simulink library "Lib_Piccolo"  (R2018b)
settings: Solver=VariableStepAuto  StartTime=0.0  StopTime=10.0  RelTol=1e-3
values from neighbouring files (symbols this model uses):
  AccelErrInt2Brakes = 0.15    [SimulationControlConfig16P.m]    (also in SimulationControlConfig16P_LEGACY.m; SimulationControlConfigTAILLESS.m = 0.2; SimulationControlConfigUTAIL.m = 0.2)
  AileronMax = 25    [SimulationControlConfig16P.m]    (also in SimulationControlConfig16P_LEGACY.m; SimulationControlConfigTAILLESS.m; SimulationControlConfigUTAIL.m)
  AileronPower = 0.00268    [SimulationControlConfig16P.m]    (also in SimulationControlConfig16P_LEGACY.m; SimulationControlConfigTAILLESS.m; SimulationControlConfigUTAIL.m)
  AileronSurfaceMax = 45    [SimulationControlConfig16P.m]    (also in SimulationControlConfig16P_LEGACY.m)
  AileronTrim = 0    [SimulationControlConfig16P.m]    (also in SimulationControlConfig16P_LEGACY.m; SimulationControlConfigTAILLESS.m; SimulationControlConfigUTAIL.m)
  Alt = 1000 + TerrainHeight    [SimulationStateConfig.m]
  AltCruise_m = testPlans(testIndx).terrainElevation * 0.3048 + 200    [SimulationControlConfig16P.m]    (also in SimulationControlConfigTAILLESS.m = 1083; SimulationControlConfigUTAIL.m = testPlans(testIndx).terrainElevation * 0.3048 + 152)
  AltitudeRate2PitchCmdIntegratorInit = 0.1    [SimulationControlPre.m]
  AltMax = 10000    [SimulationControlConfig16P.m]    (also in SimulationControlConfig16P_LEGACY.m; SimulationControlConfigTAILLESS.m; SimulationControlConfigUTAIL.m)
  AltMaxAccel = 1.25    [SimulationControlConfig16P.m]    (also in SimulationControlConfig16P_LEGACY.m = 0.9; SimulationControlConfigTAILLESS.m = 1.7; SimulationControlConfigUTAIL.m = 2)
  AltMin = 0    [SimulationControlConfig16P.m]    (also in SimulationControlConfig16P_LEGACY.m; SimulationControlConfigTAILLESS.m; SimulationControlConfigUTAIL.m)
  AltRateCmd2Pitch = 0.50    (= 0.5)    [SimulationControlConfig16P.m]    (also in SimulationControlConfig16P_LEGACY.m = 0.6; SimulationControlConfigTAILLESS.m = 0.2; SimulationControlConfigUTAIL.m = 0.3)
  AltRateError2Pitch = 0.40    (= 0.4)    [SimulationControlConfig16P.m]    (also in SimulationControlConfig16P_LEGACY.m; SimulationControlConfigTAILLESS.m = 0.55; SimulationControlConfigUTAIL.m = 0.55)
  AltRateErrorInt2Pitch = 0.50    (= 0.5)    [SimulationControlConfig16P.m]    (also in SimulationControlConfig16P_LEGACY.m = 0.45; SimulationControlConfigTAILLESS.m; SimulationControlConfigUTAIL.m = 0.75)
  AltRateLpfCutOff = 3    [SimulationControlConfig16P.m]    (also in SimulationControlConfig16P_LEGACY.m; SimulationControlConfigTAILLESS.m = 2; SimulationControlConfigUTAIL.m = 2)
  AutoNosegear2Rudder = 26    [SimulationControlConfig16P.m]    (also in SimulationControlConfig16P_LEGACY.m; SimulationControlConfigTAILLESS.m = 25.2; SimulationControlConfigUTAIL.m = 14)
  b = 5.54    [SimulationControlConfig16P.m]    (also in SimulationControlConfig16P_LEGACY.m; SimulationControlConfigTAILLESS.m = 2.37; SimulationControlConfigUTAIL.m = 2.37)
  Bank2AileronIntegratorInit = 0    [SimulationControlPre.m]
  BankMax_User = BankMax_User/180*pi    (= 0.523598775598)    [SimulationControlConfig16P.m]    (also in SimulationControlConfig16P_LEGACY.m; SimulationControlConfigTAILLESS.m = 0.610865238198; SimulationControlConfigUTAIL.m = 0.628318530718)
  baseLegFlaps = 20    [SimulationControlConfig16P.m]    (also in SimulationControlConfig16P_LEGACY.m = 0; SimulationControlConfigTAILLESS.m = 15; SimulationControlConfigUTAIL.m = 10)
  C = GeneticOpt.C    [SimulationCostFunction.m]
  c = Sw/b    (= 0.841696750903)    [SimulationControlConfig16P.m]    (also in SimulationControlConfig16P_LEGACY.m; SimulationControlConfigTAILLESS.m = 0.354008438819; SimulationControlConfigUTAIL.m = 0.354008438819)
  cell2WheelFactorMG = 5.98    [SimulationSensorConfig16P_LEGACY.m]
  cell2WheelFactorNG = 1    [SimulationSensorConfig16P_LEGACY.m]
  cellSatMaxMG = 15000    [SimulationSensorConfig16P.m]    (also in SimulationSensorConfig16P_LEGACY.m; SimulationSensorConfigTAILLESS7P.m; SimulationSensorConfigUTAIL7P.m)
  cellSatMaxNG = 1000    [SimulationSensorConfig16P.m]    (also in SimulationSensorConfig16P_LEGACY.m; SimulationSensorConfigTAILLESS7P.m; SimulationSensorConfigUTAIL7P.m)
  cellSatMinMG = -15000    [SimulationSensorConfig16P.m]    (also in SimulationSensorConfig16P_LEGACY.m; SimulationSensorConfigTAILLESS7P.m; SimulationSensorConfigUTAIL7P.m)
  cellSatMinNG = -1000    [SimulationSensorConfig16P.m]    (also in SimulationSensorConfig16P_LEGACY.m; SimulationSensorConfigTAILLESS7P.m; SimulationSensorConfigUTAIL7P.m)
  CL_Limit = CL_Max    (= 0.54)    [SimulationControlConfig16P.m]    (also in SimulationControlConfig16P_LEGACY.m; SimulationControlConfigTAILLESS.m; SimulationControlConfigUTAIL.m = 0.53)
  CL_Max = 0.54    [SimulationControlConfig16P.m]    (also in SimulationControlConfig16P_LEGACY.m; SimulationControlConfigTAILLESS.m; SimulationControlConfigUTAIL.m = 0.53)
  CL_Max_Nom = 0.465    [SimulationControlConfig16P.m]    (also in SimulationControlConfig16P_LEGACY.m; SimulationControlConfigTAILLESS.m = 0.39; SimulationControlConfigUTAIL.m)
  CL_Min = 0    [SimulationControlConfig16P.m]    (also in SimulationControlConfig16P_LEGACY.m; SimulationControlConfigTAILLESS.m; SimulationControlConfigUTAIL.m)
  ClimbMaxFraction = 0.35    [SimulationControlConfig16P.m]    (also in SimulationControlConfig16P_LEGACY.m = 0.24; SimulationControlConfigTAILLESS.m = 0.19; SimulationControlConfigUTAIL.m = 0.21)
  ClimboutMaxBank = 7.0    (= 7)    [SimulationControlConfig16P.m]    (also in SimulationControlConfig16P_LEGACY.m; SimulationControlConfigTAILLESS.m = 5; SimulationControlConfigUTAIL.m)
  ClimboutTimer = 7.0    (= 7)    [SimulationControlConfig16P.m]    (also in SimulationControlConfig16P_LEGACY.m; SimulationControlConfigTAILLESS.m; SimulationControlConfigUTAIL.m)
  dCl_per_dFlap = 0.005581818    [SimulationControlConfig16P.m]    (also in SimulationControlConfig16P_LEGACY.m = 0; SimulationControlConfigTAILLESS.m = 0; SimulationControlConfigUTAIL.m = 0)
  DecelerationCmd = 3.1    [SimulationControlConfig16P.m]    (also in SimulationControlConfig16P_LEGACY.m; SimulationControlConfigTAILLESS.m = 0.1; SimulationControlConfigUTAIL.m = 0.1)
  DeRotateLogicEndTimer = abs((NoseDownLimit_Deg-1)/DeRotateRamp_Dps)    [SimulationControlConfig16P.m]    (also in SimulationControlConfig16P_LEGACY.m; SimulationControlConfigTAILLESS.m; SimulationControlConfigUTAIL.m)
  DeRotateLogicHoldNoseUpTimer = 0.1    [SimulationControlConfig16P.m]    (also in SimulationControlConfig16P_LEGACY.m; SimulationControlConfigTAILLESS.m; SimulationControlConfigUTAIL.m)
  DeRotateLogicTimerTimeout = 2    [SimulationControlConfig16P.m]    (also in SimulationControlConfig16P_LEGACY.m; SimulationControlConfigTAILLESS.m; SimulationControlConfigUTAIL.m)
  DeRotateLowerCmdSaturation = 0    [SimulationControlConfig16P.m]    (also in SimulationControlConfig16P_LEGACY.m; SimulationControlConfigTAILLESS.m; SimulationControlConfigUTAIL.m)
  DeRotateRamp_Dps = 3    [SimulationControlConfig16P.m]    (also in SimulationControlConfig16P_LEGACY.m; SimulationControlConfigTAILLESS.m = 8; SimulationControlConfigUTAIL.m = 8)
  DeRotateUpperCmdSaturation = 7    [SimulationControlConfig16P.m]    (also in SimulationControlConfig16P_LEGACY.m; SimulationControlConfigTAILLESS.m; SimulationControlConfigUTAIL.m)
  DescentMaxFraction = 0.22    [SimulationControlConfig16P.m]    (also in SimulationControlConfig16P_LEGACY.m = 0.2; SimulationControlConfigTAILLESS.m = 0.17; SimulationControlConfigUTAIL.m = 0.17)
  DesktopSimTerrainOffset_m = 0.406    [SimulationAircraftConfig.m]
  downwindFlaps = 0    [SimulationControlConfig16P.m]    (also in SimulationControlConfig16P_LEGACY.m; SimulationControlConfigTAILLESS.m; SimulationControlConfigUTAIL.m)
  DP_init = 0.5*1.225*V_init^2    [SimulationControlConfig16P.m]    (also in SimulationControlConfig16P_LEGACY.m; SimulationControlConfigTAILLESS.m; SimulationControlConfigUTAIL.m)
  dscNoiseMG = 1    [SimulationSensorConfig16P_LEGACY.m]
  dscNoiseNG = 0.25    [SimulationSensorConfig16P_LEGACY.m]
  DSCnumBits = 24    [SimulationSensorConfig16P.m]    (also in SimulationSensorConfig16P_LEGACY.m; SimulationSensorConfigTAILLESS7P.m; SimulationSensorConfigUTAIL7P.m)
  DSCRangeMaxMG = 15000    [SimulationSensorConfig16P.m]    (also in SimulationSensorConfig16P_LEGACY.m; SimulationSensorConfigTAILLESS7P.m; SimulationSensorConfigUTAIL7P.m)
  DSCRangeMaxNG = 1000    [SimulationSensorConfig16P.m]    (also in SimulationSensorConfig16P_LEGACY.m; SimulationSensorConfigTAILLESS7P.m; SimulationSensorConfigUTAIL7P.m)
  DSCRangeMinMG = -15000    [SimulationSensorConfig16P.m]    (also in SimulationSensorConfig16P_LEGACY.m; SimulationSensorConfigTAILLESS7P.m; SimulationSensorConfigUTAIL7P.m)
  DSCRangeMinNG = -1000    [SimulationSensorConfig16P.m]    (also in SimulationSensorConfig16P_LEGACY.m; SimulationSensorConfigTAILLESS7P.m; SimulationSensorConfigUTAIL7P.m)
  dt = DLLSim.dt    [SimulationTimeStep.m]    (also in SimulationTrim.m = 0.02)
  EarlyTouchdownThreshold = 3.0    (= 3)    [SimulationControlConfig16P.m]    (also in SimulationControlConfig16P_LEGACY.m; SimulationControlConfigTAILLESS.m = 2.2; SimulationControlConfigUTAIL.m = 2.5)
  ElevatorDeflectionRate = 15    [SimulationControlConfig16P.m]    (also in SimulationControlConfig16P_LEGACY.m = 12; SimulationControlConfigTAILLESS.m = 10; SimulationControlConfigUTAIL.m = 12)
  ElevatorMax = 25    [SimulationControlConfig16P.m]    (also in SimulationControlConfig16P_LEGACY.m; SimulationControlConfigTAILLESS.m; SimulationControlConfigUTAIL.m)
  ElevatorPower = -0.002209    [SimulationControlConfig16P.m]    (also in SimulationControlConfig16P_LEGACY.m; SimulationControlConfigTAILLESS.m = -0.002956; SimulationControlConfigUTAIL.m = -0.00205983)
  ElevatorTrim = -3.5    [SimulationControlConfig16P.m]    (also in SimulationControlConfig16P_LEGACY.m; SimulationControlConfigTAILLESS.m = -6; SimulationControlConfigUTAIL.m = -8)
  elevonBias = 0    [SimulationControlConfig16P.m]    (also in SimulationControlConfig16P_LEGACY.m; SimulationControlConfigTAILLESS.m; SimulationControlConfigUTAIL.m)
  Enable_TAS_Protection = 0    [SimulationControlConfig16P.m]    (also in SimulationControlConfig16P_LEGACY.m; SimulationControlConfigTAILLESS.m; SimulationControlConfigUTAIL.m)
  EnableCrossTrackAbort = 1    [SimulationControlConfig16P.m]    (also in SimulationControlConfigTAILLESS.m; SimulationControlConfigUTAIL.m)
  EnergyBandwidth = 0.02    [SimulationControlConfig16P.m]    (also in SimulationControlConfig16P_LEGACY.m; SimulationControlConfigTAILLESS.m = 0.06; SimulationControlConfigUTAIL.m = 0.06)
  EngineLhFuelCut = 0    [SimulationAircraftConfig.m]
  EngineRhFuelCut = 0    [SimulationAircraftConfig.m]
  FastThrottleRate = 0.075    [SimulationControlConfig16P.m]    (also in SimulationControlConfig16P_LEGACY.m = 0.05; SimulationControlConfigTAILLESS.m = 0.1; SimulationControlConfigUTAIL.m = 0.1)
  FilterWarmUpTime = 2    [SimulationSensorConfig16P.m]    (also in SimulationSensorConfig16P_LEGACY.m; SimulationSensorConfigTAILLESS7P.m; SimulationSensorConfigUTAIL7P.m)
  finalApproachFlaps = 20    [SimulationControlConfig16P.m]    (also in SimulationControlConfig16P_LEGACY.m = 0; SimulationControlConfigTAILLESS.m = 22; SimulationControlConfigUTAIL.m = 10)
  FinalDescentSlope_Deg = testPlans(testIndx).descentSlope    [SimulationControlConfig16P.m]    (also in SimulationControlConfig16P_LEGACY.m; SimulationControlConfigTAILLESS.m; SimulationControlConfigUTAIL.m)
  flapMax = 0    [SimulationControlConfig16P.m]    (also in SimulationControlConfig16P_LEGACY.m; SimulationControlConfigTAILLESS.m; SimulationControlConfigUTAIL.m)
  flapRate = 7.5    [SimulationControlConfig16P.m]    (also in SimulationControlConfig16P_LEGACY.m; SimulationControlConfigTAILLESS.m = 6.6; SimulationControlConfigUTAIL.m)
  FlareHeight = 5    [SimulationControlConfig16P.m]    (also in SimulationControlConfig16P_LEGACY.m = 4.8; SimulationControlConfigTAILLESS.m = 2.5; SimulationControlConfigUTAIL.m = 2)
  FlareVerticalRate_mps = -0.4    [SimulationControlConfig16P.m]    (also in SimulationControlConfig16P_LEGACY.m = -0.5; SimulationControlConfigTAILLESS.m = -0.15; SimulationControlConfigUTAIL.m = -0.15)
  Fp_Aileron = 0.55*2*pi*RollRateLpfCutoff*dt    [SimulationControlConfig16P.m]    (also in SimulationControlConfig16P_LEGACY.m; SimulationControlConfigTAILLESS.m; SimulationControlConfigUTAIL.m)
  Fp_Alt = 0.55*AltBandwidth    (= 0.099)    [SimulationControlConfig16P.m]    (also in SimulationControlConfig16P_LEGACY.m; SimulationControlConfigTAILLESS.m = 0.587477826221; SimulationControlConfigUTAIL.m = 0.69115038379)
  Fp_AltRate = 0.55*2*pi*AltRateLpfCutOff*dt    [SimulationControlConfig16P.m]    (also in SimulationControlConfig16P_LEGACY.m; SimulationControlConfigTAILLESS.m; SimulationControlConfigUTAIL.m)
  Fp_Elevator = 0.55*2*pi*PitchRateLpfCutoff*dt    [SimulationControlConfig16P.m]    (also in SimulationControlConfig16P_LEGACY.m; SimulationControlConfigTAILLESS.m; SimulationControlConfigUTAIL.m)
  Fp_Energy = 0.55*2*pi*EnergyBandwidth    (= 0.069115038379)    [SimulationControlConfig16P.m]    (also in SimulationControlConfig16P_LEGACY.m; SimulationControlConfigTAILLESS.m = 0.207345115137; SimulationControlConfigUTAIL.m = 0.207345115137)
  Fp_Energy2 = 0.55*2*pi*EnergyBandwidth*dt    [SimulationControlConfig16P.m]    (also in SimulationControlConfig16P_LEGACY.m; SimulationControlConfigTAILLESS.m; SimulationControlConfigUTAIL.m)
  Fp_Pitch = 0.55*2*pi*PitchBandwidth    (= 2.76460153516)    [SimulationControlConfig16P.m]    (also in SimulationControlConfig16P_LEGACY.m = 3.11017672705; SimulationControlConfigTAILLESS.m = 3.80132711084; SimulationControlConfigUTAIL.m = 2.41902634326)
  Fp_Pitch_2 = 0.55*2*pi*PitchBandwidth*dt    [SimulationControlConfig16P.m]    (also in SimulationControlConfig16P_LEGACY.m; SimulationControlConfigTAILLESS.m; SimulationControlConfigUTAIL.m)
  Fp_Roll = RollBandwidth^2    (= 1)    [SimulationControlConfig16P.m]    (also in SimulationControlConfig16P_LEGACY.m = 1.44; SimulationControlConfigTAILLESS.m; SimulationControlConfigUTAIL.m)
  Fp_Rudder = 0.55*2*pi*YawRateLpfCutoff*dt    [SimulationControlConfig16P.m]    (also in SimulationControlConfig16P_LEGACY.m; SimulationControlConfigTAILLESS.m; SimulationControlConfigUTAIL.m)
  Fp_TAS = 0.55*2*pi*TASBandwidth    (= 0.103672557568)    [SimulationControlConfig16P.m]    (also in SimulationControlConfig16P_LEGACY.m; SimulationControlConfigTAILLESS.m = 0.172787595947; SimulationControlConfigUTAIL.m = 0.172787595947)
  Fp_TAS_Filter = 2*pi*TasLpfCutoff*dt    [SimulationControlConfig16P.m]    (also in SimulationControlConfig16P_LEGACY.m; SimulationControlConfigTAILLESS.m; SimulationControlConfigUTAIL.m)
  Fp_Turn = 0.55*2*pi*TurnErrLPFcutoff    (= 0.0345575191895)    [SimulationControlConfig16P.m]    (also in SimulationControlConfig16P_LEGACY.m; SimulationControlConfigTAILLESS.m = 0.172787595947; SimulationControlConfigUTAIL.m = 0.172787595947)
  Fp_TurnDerr = 0.55*2*pi*TurnDerivativeLPFcutoff    (= 0.0345575191895)    [SimulationControlConfig16P.m]    (also in SimulationControlConfig16P_LEGACY.m; SimulationControlConfigTAILLESS.m = 0.172787595947; SimulationControlConfigUTAIL.m = 0.172787595947)
  FTV = 3    [SimulationAircraftConfig.m]
  ftvStaticPositionError = 1/1.18    (= 0.847457627119)    [SimulationSensorConfig16P.m]    (also in SimulationSensorConfig16P_LEGACY.m; SimulationSensorConfigTAILLESS7P.m = 1; SimulationSensorConfigUTAIL7P.m = 1)
  g = 9.81    [SimulationStateConfig.m]
  GustSpd_Kts = testPlans(testIndx).gustSpd    [SimulationStateConfig.m]
  GustTriggerVal = testPlans(testIndx).gustTriggerVal    [SimulationStateConfig.m]
  HeadingErr2TurnRate = 0.5    [SimulationControlConfig16P.m]    (also in SimulationControlConfig16P_LEGACY.m; SimulationControlConfigTAILLESS.m; SimulationControlConfigUTAIL.m)
  HeadingErrDer2TurnRate = 0.3    [SimulationControlConfig16P.m]    (also in SimulationControlConfig16P_LEGACY.m; SimulationControlConfigTAILLESS.m; SimulationControlConfigUTAIL.m)
  IASbounce = IASstall*0.8    [SimulationControlPre.m]
  IAScruiseCMD = sqrt(2*m*9.81/(1.225*Sw*CL_cruise))    [SimulationControlConfig16P.m]    (also in SimulationControlConfig16P_LEGACY.m; SimulationControlConfigTAILLESS.m; SimulationControlConfigUTAIL.m)
  IASfinalCMD = 1.12 * IASmin    [SimulationControlConfig16P.m]    (also in SimulationControlConfig16P_LEGACY.m = 1.10 * IASmin; SimulationControlConfigTAILLESS.m = 1.10 * IASmin; SimulationControlConfigUTAIL.m = 1.15 * IASmin)
  IASflareCMD = IASstall    [SimulationControlConfig16P.m]    (also in SimulationControlConfig16P_LEGACY.m; SimulationControlConfigTAILLESS.m; SimulationControlConfigUTAIL.m)
  IASmax = 64    [SimulationControlConfig16P.m]    (also in SimulationControlConfig16P_LEGACY.m = 46; SimulationControlConfigTAILLESS.m = 38.58; SimulationControlConfigUTAIL.m = 35)
  IASmin = sqrt(2*m*9.81/(1.225*Sw*0.9*CL_Max_Nom))    [SimulationControlConfig16P.m]    (also in SimulationControlConfig16P_LEGACY.m; SimulationControlConfigTAILLESS.m; SimulationControlConfigUTAIL.m)
  IASshortCMD = IASstall    [SimulationControlConfig16P.m]    (also in SimulationControlConfig16P_LEGACY.m; SimulationControlConfigTAILLESS.m; SimulationControlConfigUTAIL.m)
  IASstall = sqrt(2*m*9.81/(1.225*Sw*CL_Max))    [SimulationControlConfig16P.m]    (also in SimulationControlConfig16P_LEGACY.m; SimulationControlConfigTAILLESS.m; SimulationControlConfigUTAIL.m)
  inFlight = 1    [SimulationControlConfig16P.m]    (also in SimulationControlConfigTAILLESS.m; SimulationControlConfigUTAIL.m)
  JetCatOffset = 5    [SimulationControlConfig16P.m]    (also in SimulationControlConfig16P_LEGACY.m)
  LaunchRollingElevator = -1.5    [SimulationControlConfig16P.m]    (also in SimulationControlConfig16P_LEGACY.m; SimulationControlConfigTAILLESS.m = 1; SimulationControlConfigUTAIL.m = 1)
  ldg_NosegearMax = 10    [SimulationControlConfig16P.m]    (also in SimulationControlConfig16P_LEGACY.m; SimulationControlConfigTAILLESS.m; SimulationControlConfigUTAIL.m)
  ldg_TrackVyErrInt2Nosegear = 0.1250    (= 0.125)    [SimulationControlConfig16P.m]    (also in SimulationControlConfig16P_LEGACY.m; SimulationControlConfigTAILLESS.m = 0.00714285714286; SimulationControlConfigUTAIL.m = 0.00714285714286)
  ldg_TrackVyErrPro2Nosegear = 0.35    [SimulationControlConfig16P.m]    (also in SimulationControlConfig16P_LEGACY.m; SimulationControlConfigTAILLESS.m = 0.0546666666667; SimulationControlConfigUTAIL.m = 0.0546666666667)
  ldg_TrackY2Vy = 0.07    [SimulationControlConfig16P.m]    (also in SimulationControlConfig16P_LEGACY.m; SimulationControlConfigTAILLESS.m = 0.17; SimulationControlConfigUTAIL.m = 0.17)
  ldg_Vy2NosegearScalingPower = 1.075    [SimulationControlConfig16P.m]    (also in SimulationControlConfig16P_LEGACY.m; SimulationControlConfigTAILLESS.m = 0.6; SimulationControlConfigUTAIL.m = 0.5)
  ldg_Y2VyScalingPower = 0.175    [SimulationControlConfig16P.m]    (also in SimulationControlConfig16P_LEGACY.m; SimulationControlConfigTAILLESS.m = 0; SimulationControlConfigUTAIL.m = 0)
  ldg_YawRate2Nosegear = 0.175    [SimulationControlConfig16P.m]    (also in SimulationControlConfig16P_LEGACY.m; SimulationControlConfigTAILLESS.m = 0.065; SimulationControlConfigUTAIL.m = 0.065)
  LiftSlope = 0.064285    [SimulationControlConfig16P.m]    (also in SimulationControlConfig16P_LEGACY.m; SimulationControlConfigTAILLESS.m = 0.058631; SimulationControlConfigUTAIL.m)
  LPFaileronInit = 0    [SimulationControlPre.m]
  LPFclestInit = 0    [SimulationControlPre.m]
  LPFenergyFFInit = 0    [SimulationControlPre.m]
  LPFtasInit = V_init + 2    [SimulationControlPre.m]
  LPFthrottleInit = ThrottleTrim    [SimulationControlPre.m]
  LPFturnErrInit = 0    [SimulationControlPre.m]
  ... (+115 more)
undefined symbols (not defined in the file or in its folder): abortFlag, alphaHPF, apmDelay, BRWNOUT, CRAWOR, CRAWUR, DiscIntNeverNeededParam, DLLSim, DLLSimStep, ECOMOR, ECOMUR, Fp_Tas, GustTrigger_HeightAgl_m, IPSTAT, LCINTEG, Ldg_Persist_Time, LOWER_FLAGS, MSG_ENABLE, NoiseStd, OLDVAL, OVERRIDE_ENABLE, OVERRIDE_VALUE, REBOOT, reversionEnable, revIASMax, revIASMin, revPitchMax, revPitchMin, revPitchRateMax, revRollMax, revRollRateMax, SAMPLE, SCALON, SensorModel, sigbuilder_block, Sim_Vx, Sim_Vy, Sim_Vz, Sim_Xpos, Sim_Ypos, Sim_Zpos, SYSOR, SYSUR, TARE, TEMPOR, TEMPUR, testIndx, testPlan, testPlans, Trim_piccoloInCmd, Trim_REFSI_FD_IN_nmodeCgShifterCmd_Ft, Trim_REFSI_FD_IN_nmodeFlapLhIBCmd_Deg, Trim_REFSI_FD_IN_nmodeFlapLhOBCmd_Deg, Trim_REFSI_FD_IN_nmodeFlapRhIBCmd_Deg, Trim_REFSI_FD_IN_nmodeFlapRhOBCmd_Deg, Trim_REFSI_FD_IN_nmodeSlatLhCmd_Deg, Trim_REFSI_FD_IN_nmodeSlatRhCmd_Deg, Trim_REFSI_FD_IN_nmodeSplrLhInbdCmd_Deg, Trim_REFSI_FD_IN_nmodeSplrLhOutbdCmd_Deg ... (+5)
libraries: simulink x866, aerolibconvert2 x60, $bdroot x52, aerolibatmos2 x5, dspswit3 x5, simulink_extras x4, dsparch4 x2, Lib_Piccolo_Alt x2, eeGeneralControl x1, dspindex x1
(part 22 of 44)

== system Lib_Piccolo/Pitch to Elevator/1st Order Reference Model/PitchRate Max Accel Limit ==
  note: U(k)
  note: Y(k)
  up : Inport
  u : Inport  Port=2
  lo : Inport  Port=3
  Delay Input2 : UnitDelay  Description=Store in Global RAM  DisableCoverage=on  InitialCondition=RateLimitPitchRateAccel  SampleTime=-1
  Difference Inputs1 : Sum  Description=Add in CPU  DisableCoverage=on  Inputs=+-  OutDataTypeStr=Inherit: Inherit via back propagation
  Difference Inputs2 : Sum  Description=Add in CPU  OutDataTypeStr=Inherit: Inherit via back propagation
  FixPt Data Type Duplicate : DataTypeDuplicate  DisableCoverage=on  NumInputPorts=7
  Flagged Saturation : $bdroot/Pitch to Elevator/1st Order Reference Model/PitchRateCMD Limit  SystemSampleTime=-1
  delta fall limit : Product  DisableCoverage=on  Inputs=**  OutDataTypeStr=Inherit: Inherit via back propagation  SaturateOnIntegerOverflow=on
  delta rise limit : Product  DisableCoverage=on  Inputs=**  OutDataTypeStr=Inherit: Inherit via back propagation  SaturateOnIntegerOverflow=on
  sample time : SampleTimeMath  DisableCoverage=on  TsampMathOp=Ts Only  weightValue=1
  Y : Outport  InitialOutput=0
  upperFlag : Outport  Port=2
  lowerFlag : Outport  Port=3
  wires:
  delta fall limit/1 -> Flagged Saturation/3, FixPt Data Type Duplicate/3
  Difference Inputs1/1 -> Flagged Saturation/2, FixPt Data Type Duplicate/4  "( U(k) - Y(k-1) )"
  delta rise limit/1 -> FixPt Data Type Duplicate/6, Flagged Saturation/1
  lo/1 -> delta fall limit/1
  Flagged Saturation/3 -> FixPt Data Type Duplicate/7, Difference Inputs2/1
  u/1 -> Difference Inputs1/1, FixPt Data Type Duplicate/5, sample time/1
  up/1 -> delta rise limit/1
  Delay Input2/1 -> Difference Inputs2/2, Difference Inputs1/2, FixPt Data Type Duplicate/2  "Y(k-1)"
  sample time/1 -> delta fall limit/2, delta rise limit/2
  Difference Inputs2/1 -> Delay Input2/1, FixPt Data Type Duplicate/1, Y/1
  Flagged Saturation/1 -> upperFlag/1
  Flagged Saturation/2 -> lowerFlag/1

== system Lib_Piccolo/Pitch to Elevator/1st Order Reference Model/PitchRateCMD Limit ==
  up : Inport
  u : Inport  Port=2
  lo : Inport  Port=3
  Data Type Duplicate : DataTypeDuplicate  DisableCoverage=on
  Data Type Propagation : simulink/Signal Attributes/Data Type Propagation  PropDataType=fixdt(1, 16)  IfRefDouble=double  IfRefSingle=single  IsSigned=IsSigned1  NumBitsBase=NumBits1  NumBitsMult=1  NumBitsAdd=0  NumBitsAllowFinal=1:128  PropScaling=2^-10  ValuesUsedBestPrec=[5 -7]  SlopeBase=Slope1  SlopeMult=1  SlopeAdd=0  BiasBase=Bias1  BiasMult=1  BiasAdd=0
      settings: SourceProductName=Simulink  SourceProductBaseCode=SL
  LowerRelop1 : RelationalOperator  DisableCoverage=on  Operator=>  OutDataTypeStr=boolean  RndMeth=Nearest
  Switch : Switch  Criteria=u2 ~= 0  OutDataTypeStr=Inherit: Inherit via back propagation  ZeroCross=off
  Switch2 : Switch  Criteria=u2 ~= 0  OutDataTypeStr=Inherit: Inherit via back propagation  ZeroCross=off
  UpperRelop : RelationalOperator  DisableCoverage=on  Operator=<  OutDataTypeStr=boolean  RndMeth=Nearest
  upperFlag : Outport
  lowerFlag : Outport  Port=2
  y : Outport  Port=3
  wires:
  UpperRelop/1 -> Switch/2, upperFlag/1
  Switch/1 -> Data Type Duplicate/2, Switch2/3, Data Type Propagation/3
  LowerRelop1/1 -> Switch2/2, lowerFlag/1
  lo/1 -> Switch/1, UpperRelop/2
  u/1 -> Data Type Propagation/2, Data Type Propagation/1, LowerRelop1/1, Switch/3, UpperRelop/1
  Switch2/1 -> Data Type Duplicate/1, y/1
  up/1 -> Switch2/1, LowerRelop1/2

== system Lib_Piccolo/Pitch to Elevator/1st Order Reference Model/resetCondition ==
  apMode : Inport
  Compare To Constant1 : simulink/Logic and Bit Operations/Compare To Constant  relop=<=  const=2  OutDataTypeStr=uint8
  Compare To Constant3 : simulink/Logic and Bit Operations/Compare To Constant  relop===  const=11  OutDataTypeStr=uint8
  NOT : Logic  Operator=NOT  IconShape=distinctive  AllPortsSameDT=off  OutDataTypeStr=boolean
  OR : Logic  Operator=OR  Inputs=3  IconShape=distinctive  AllPortsSameDT=off  OutDataTypeStr=boolean
  Reset : Outport
  wires:
  NOT/1 -> OR/3
  [ApGlobal] -> NOT/1
  Compare To Constant1/1 -> OR/2
  OR/1 -> Reset/1
  Compare To Constant3/1 -> OR/1
  apMode/1 -> Compare To Constant3/1, Compare To Constant1/1

== system Lib_Piccolo/Pitch to Elevator/Cm//Alpha Estimation/LPF CLest ==
  Input : Inport
  Reset : Inport  Port=2
  Add1 : Sum  Inputs=++|
  Compare To Constant2 : simulink/Logic and Bit Operations/Compare To Constant  relop=>  const=0  OutDataTypeStr=uint8
  Constant11 : Constant  Value=PitchBandwidth
  "LPF " : DiscreteTransferFcn  Commented=on  Numerator=[(2*Fp_Pitch_2) 0]  Denominator=[1 (2*Fp_Pitch_2-1)]  InitialStates=3
  Switch1 : Switch  Criteria=u2 > Threshold
  Unit Delay1 : UnitDelay  InitialCondition=LPFclestInit  SampleTime=-1
  a1 : Gain  Gain=1-(2*Fp_Pitch_2)
  b0 : Gain  Gain=(2*Fp_Pitch_2)
  Output : Outport
  wires:
  Unit Delay1/1 -> a1/1
  b0/1 -> Add1/2
  a1/1 -> Add1/1
  Add1/1 -> Unit Delay1/1, Switch1/1
  Input/1 -> Switch1/3, b0/1
  Switch1/1 -> Output/1
  Compare To Constant2/1 -> Switch1/2
  Constant11/1 -> Compare To Constant2/1

== system Lib_Piccolo/Pitch to Elevator/DynamicPLimit/Latch ==
  D : Inport
  Enable/!Rst : Inport  Port=2
  AND : Logic  IconShape=distinctive  AllPortsSameDT=off  OutDataTypeStr=boolean
  Constant : Constant
  OR : Logic  Operator=OR  IconShape=distinctive  AllPortsSameDT=off  OutDataTypeStr=boolean
  Switch : Switch  Criteria=u2 > Threshold  Threshold=0.5
  Unit Delay : UnitDelay  SampleTime=-1
  Q_Latched : Outport
  wires:
  Constant/1 -> Switch/1
  Enable/!Rst/1 -> AND/2
  AND/1 -> Switch/2
  OR/1 -> AND/1
  D/1 -> OR/1, Switch/3
  Switch/1 -> Unit Delay/1, Q_Latched/1
  Unit Delay/1 -> OR/2

== system Lib_Piccolo/Pitch to Elevator/Elevator Ramp Logic/Elevator DeRotation Ramp ==
  Elevator In : Inport
  apMode In : Inport  Port=2
  Compare To Constant2 : simulink/Logic and Bit Operations/Compare To Constant  relop===  const=11  OutDataTypeStr=uint8
  Constant : Constant  Value=ElevatorDeflectionRate
  Discrete-Time Integrator : DiscreteIntegrator  ExternalReset=rising  InitialConditionSource=external  SampleTime=-1  LimitOutput=on  UpperSaturationLimit=RollingElevator  LowerSaturationLimit=-ElevatorMax  ICPrevOutput=DiscIntNeverNeededParam  ICPrevScaledInput=DiscIntNeverNeededParam
  NOT : Logic  Operator=NOT  IconShape=distinctive  AllPortsSameDT=off  OutDataTypeStr=boolean
  Switch : Switch  Criteria=u2 > Threshold
  Unit Delay : UnitDelay  SampleTime=-1
  Elevator Out : Outport
  wires:
  Compare To Constant2/1 -> NOT/1, Discrete-Time Integrator/2
  apMode In/1 -> Compare To Constant2/1
  Unit Delay/1 -> Discrete-Time Integrator/3
  Switch/1 -> Elevator Out/1
  NOT/1 -> Switch/2
  Elevator In/1 -> Switch/1, Unit Delay/1
  Constant/1 -> Discrete-Time Integrator/1
  Discrete-Time Integrator/1 -> Switch/3  "Sim.rampElevator"

== system Lib_Piccolo/Pitch to Elevator/Elevator Ramp Logic/Elevator Rotation Ramp ==
  Elevator In : Inport
  apMode In : Inport  Port=2
  Compare To Constant2 : simulink/Logic and Bit Operations/Compare To Constant  relop===  const=2  OutDataTypeStr=uint8
  Constant : Constant  Value=RotationRate
  Constant1 : Constant  Value=LaunchRollingElevator
  Constant2 : Constant  Value=LaunchRollingElevator
  Discrete-Time Integrator : DiscreteIntegrator  ExternalReset=rising  InitialConditionSource=external  SampleTime=-1  LimitOutput=on  UpperSaturationLimit=LaunchRollingElevator  LowerSaturationLimit=RotationElevator  ICPrevOutput=DiscIntNeverNeededParam  ICPrevScaledInput=DiscIntNeverNeededParam
  NOT : Logic  Operator=NOT  IconShape=distinctive  AllPortsSameDT=off  OutDataTypeStr=boolean
  Switch : Switch  Criteria=u2 > Threshold
  Switch1 : Switch  Threshold=2
  Elevator Out : Outport
  wires:
  Constant1/1 -> Switch1/3
  Switch1/1 -> Elevator Out/1
  Switch/1 -> Switch1/1
  Compare To Constant2/1 -> NOT/1, Discrete-Time Integrator/2
  apMode In/1 -> Compare To Constant2/1, Switch1/2
  Constant2/1 -> Discrete-Time Integrator/3
  NOT/1 -> Switch/2
  Elevator In/1 -> Switch/1
  Constant/1 -> Discrete-Time Integrator/1
  Discrete-Time Integrator/1 -> Switch/3  "Sim.RotationRampElevator"

== system Lib_Piccolo/Pitch to Elevator/Reference Frame Conversion and Pitch Rate Limit Determination/AeroVsStruct_Limit ==
  Q : Inport
  Compare To Constant1 : simulink/Logic and Bit Operations/Compare To Constant  Commented=on  relop=>=  const=6  OutDataTypeStr=uint8
  Compare To Constant3 : simulink/Logic and Bit Operations/Compare To Constant  Commented=on  relop=>=  const=8  OutDataTypeStr=uint8
  Constant : Constant  Value=Sw
  Constant1 : Constant  Value=CL_Limit
  Constant2 : Constant  Value=m
  Constant3 : Constant  Value=nMax_User
  Constant4 : Constant  Value=nMin_User
  Constant5 : Constant  Value=CL_Min
  Constant7 : Constant  Commented=on  Value=CL_Limit
  Constant8 : Constant  Commented=on  Value=CL_Max_Nom
  Constant9 : Constant  Commented=on  Value=CL_Limit
  Flap Compensation : Subsystem
  "Load Factors (nMax,nMin) at current conditions " : MATLAB Function  TreatAsAtomicUnit=on
  Switch : Switch  Commented=on  Criteria=u2 > Threshold
  Switch2 : Switch  Commented=on  Criteria=u2 > Threshold
  nMax : Outport
  "nMin " : Outport  Port=2
  wires:
  Flap Compensation/1(CL_Limit_adjusted) -> "Load Factors (nMax,nMin) at current conditions "/3(CL_Limit)
  Constant1/1 -> Flap Compensation/1(CL_Limit_in)
  "Load Factors (nMax,nMin) at current conditions "/2(nMin) -> "nMin "/1
  Constant5/1 -> "Load Factors (nMax,nMin) at current conditions "/4(CL_Min)
  Constant4/1 -> "Load Factors (nMax,nMin) at current conditions "/7(nMin_User)
  Constant3/1 -> "Load Factors (nMax,nMin) at current conditions "/6(nMax_User)
  Constant2/1 -> "Load Factors (nMax,nMin) at current conditions "/5(m)
  Constant/1 -> "Load Factors (nMax,nMin) at current conditions "/2(Sw)
  "Load Factors (nMax,nMin) at current conditions "/1(nMax) -> nMax/1
  Q/1 -> "Load Factors (nMax,nMin) at current conditions "/1(Q)
  Compare To Constant3/1 -> Switch2/2
  Constant8/1 -> Switch/1
  Constant7/1 -> Switch2/1
  Compare To Constant1/1 -> Switch/2
  Switch/1 -> Switch2/3
  Switch2/1 -> ?
  Constant9/1 -> Switch/3

== system Lib_Piccolo/Pitch to Elevator/TASLimit/Latch ==
  D : Inport
  Enable/!Rst : Inport  Port=2
  AND : Logic  IconShape=distinctive  AllPortsSameDT=off  OutDataTypeStr=boolean
  Constant : Constant
  OR : Logic  Operator=OR  IconShape=distinctive  AllPortsSameDT=off  OutDataTypeStr=boolean
  Switch : Switch  Criteria=u2 > Threshold  Threshold=0.5
  Unit Delay : UnitDelay  SampleTime=-1
  Q_Latched : Outport
  wires:
  Constant/1 -> Switch/1
  Enable/!Rst/1 -> AND/2
  AND/1 -> Switch/2
  OR/1 -> AND/1
  D/1 -> OR/1, Switch/3
  Switch/1 -> Unit Delay/1, Q_Latched/1
  Unit Delay/1 -> OR/2

== system Lib_Piccolo/Throttle Control (Airspeed Mode)/1st Order Reference Model/Subsystem ==
  V : Inport
  Vcmd : Inport  Port=2
  "ClimbMaxFraction " : Gain  Gain=ClimbMaxFraction
  Constant : Constant  Value=IASmin
  "DescentMaxFraction " : Gain  Gain=DescentMaxFraction
  Gain : Gain  Gain=-0.3
  Gain1 : Gain  Gain=-1
  Min : MinMax  Inputs=2
  Saturation Dynamic : simulink/Discontinuities/Saturation Dynamic  OutMin=[]  OutMax=[]  OutDataTypeStr=Inherit: Same as second input  OutDataType=fixdt(1, 16)  OutScaling=2^-10  DoSatur=off
  Simplified here; should adjust based on air density : Gain
  hdotMax : Outport
  "hdotMin " : Outport  Port=2
  wires:
  Saturation Dynamic/1 -> "DescentMaxFraction "/1, "ClimbMaxFraction "/1  "V_Prime"
  "ClimbMaxFraction "/1 -> hdotMax/1
  Vcmd/1 -> Saturation Dynamic/1
  V/1 -> Gain/1, Saturation Dynamic/2
  Constant/1 -> Simplified here; should adjust based on air density/1
  Simplified here; should adjust based on air density/1 -> Saturation Dynamic/3
  Min/1 -> "hdotMin "/1
  Gain/1 -> Min/2
  "DescentMaxFraction "/1 -> Gain1/1
  Gain1/1 -> Min/1

== system Lib_Piccolo/Throttle Control (Airspeed Mode)/Subsystem/LPF Throttle Alpha ==
  Input : Inport
  Reset : Inport  Port=2
  Compare To Constant1 : simulink/Logic and Bit Operations/Compare To Constant  relop=>  const=0  OutDataTypeStr=uint8
  Constant : Constant  Value=dt
  Constant1 : Constant  Value=ThrottleLpfCutoff
  LPF Alpha Throttle : MATLAB Function  TreatAsAtomicUnit=on
  Memory1 : Memory  InitialCondition=LPFthrottleInit  InheritSampleTime=on  LinearizeAsDelay=on
  Switch : Switch  Criteria=u2 > Threshold
  Switch2 : Switch  Criteria=u2 > Threshold
  Output : Outport
  wires:
  Constant1/1 -> LPF Alpha Throttle/4(bandwidth), Compare To Constant1/1
  Memory1/1 -> LPF Alpha Throttle/1(xFiltOld)
  LPF Alpha Throttle/1(xFilt) -> Switch/3, Switch2/1
  Compare To Constant1/1 -> Switch2/2
  Input/1 -> Switch2/3, Switch/1, LPF Alpha Throttle/3(xNew)
  Switch2/1 -> Output/1
  Constant/1 -> LPF Alpha Throttle/2(dt)
  Reset/1 -> Switch/2
  Switch/1 -> Memory1/1

== system Lib_Piccolo/Throttle Control (Alt Mode)/1st Order Reference Model/TEC Ref Max Rate Limit ==
  note: Y(k)
  note: U(k)
  up : Inport
  u : Inport  Port=2
  lo : Inport  Port=3
  Delay Input2 : UnitDelay  Description=Store in Global RAM  DisableCoverage=on  SampleTime=-1
  Difference Inputs1 : Sum  Description=Add in CPU  DisableCoverage=on  Inputs=+-  OutDataTypeStr=Inherit: Inherit via back propagation
  Difference Inputs2 : Sum  Description=Add in CPU  OutDataTypeStr=Inherit: Inherit via back propagation
  FixPt Data Type Duplicate : DataTypeDuplicate  DisableCoverage=on  NumInputPorts=7
  Saturation Dynamic2 : simulink/Discontinuities/Saturation Dynamic  OutMin=[]  OutMax=[]  OutDataTypeStr=Inherit: Same as second input  OutDataType=fixdt(1, 16)  OutScaling=2^-10  DoSatur=off
  delta fall limit : Product  DisableCoverage=on  Inputs=**  OutDataTypeStr=Inherit: Inherit via back propagation  SaturateOnIntegerOverflow=on
  delta rise limit : Product  DisableCoverage=on  Inputs=**  OutDataTypeStr=Inherit: Inherit via back propagation  SaturateOnIntegerOverflow=on
  sample time : SampleTimeMath  DisableCoverage=on  TsampMathOp=Ts Only  weightValue=1
  Y : Outport  InitialOutput=0
  wires:
  Difference Inputs2/1 -> Y/1, FixPt Data Type Duplicate/1, Delay Input2/1
  sample time/1 -> delta rise limit/2, delta fall limit/2
  Delay Input2/1 -> FixPt Data Type Duplicate/2, Difference Inputs1/2, Difference Inputs2/2  "Y(k-1)"
  up/1 -> delta rise limit/1
  u/1 -> sample time/1, FixPt Data Type Duplicate/5, Difference Inputs1/1
  Saturation Dynamic2/1 -> FixPt Data Type Duplicate/7, Difference Inputs2/1
  lo/1 -> delta fall limit/1
  delta rise limit/1 -> Saturation Dynamic2/1, FixPt Data Type Duplicate/6
  Difference Inputs1/1 -> Saturation Dynamic2/2, FixPt Data Type Duplicate/4  "( U(k) - Y(k-1) )"
  delta fall limit/1 -> Saturation Dynamic2/3, FixPt Data Type Duplicate/3

== system Lib_Piccolo/Throttle Control (Alt Mode)/Filter and Throttle Cut/LPF Throttle Alpha ==
  Input : Inport
  Reset : Inport  Port=2
  Compare To Constant1 : simulink/Logic and Bit Operations/Compare To Constant  relop=>  const=0  OutDataTypeStr=uint8
  Constant : Constant  Value=dt
  Constant1 : Constant  Value=ThrottleLpfCutoff
  LPF Alpha Throttle : MATLAB Function  TreatAsAtomicUnit=on
  Memory1 : Memory  InitialCondition=LPFthrottleInit  InheritSampleTime=on  LinearizeAsDelay=on
  Switch : Switch  Criteria=u2 > Threshold
  Switch2 : Switch  Criteria=u2 > Threshold
  Output : Outport
  wires:
  Constant1/1 -> LPF Alpha Throttle/4(bandwidth), Compare To Constant1/1
  Memory1/1 -> LPF Alpha Throttle/1(xFiltOld)
  LPF Alpha Throttle/1(xFilt) -> Switch/3, Switch2/1
  Compare To Constant1/1 -> Switch2/2
  Input/1 -> Switch2/3, Switch/1, LPF Alpha Throttle/3(xNew)
  Switch2/1 -> Output/1
  Constant/1 -> LPF Alpha Throttle/2(dt)
  Reset/1 -> Switch/2
  Switch/1 -> Memory1/1

== system Lib_Piccolo/Throttle Control (Alt Mode)/Flare Throttle Modifications 2/Latch ==
  D : Inport
  Enable/!Rst : Inport  Port=2
  AND : Logic  IconShape=distinctive  AllPortsSameDT=off  OutDataTypeStr=boolean
  Constant : Constant  OutDataTypeStr=boolean
  OR : Logic  Operator=OR  IconShape=distinctive  AllPortsSameDT=off  OutDataTypeStr=boolean
  Switch : Switch  Criteria=u2 > Threshold  Threshold=0.5
  Unit Delay : UnitDelay  SampleTime=-1
  Q_Latched : Outport
  wires:
  Unit Delay/1 -> OR/2
  Switch/1 -> Q_Latched/1, Unit Delay/1
  D/1 -> Switch/3, OR/1
  OR/1 -> AND/1
  AND/1 -> Switch/2
  Enable/!Rst/1 -> AND/2
  Constant/1 -> Switch/1

== system Lib_Piccolo/Throttle Control (Alt Mode)/Flare Throttle Modifications 2/Rate Limiter ==
  note: U(k)
  note: Y(k)
  up : Inport
  u : Inport  Port=2
  lo : Inport  Port=3
  Enable : Inport  Port=4
  AND : Logic  Commented=on  IconShape=distinctive  AllPortsSameDT=off  OutDataTypeStr=boolean
  Delay Input2 : UnitDelay  Description=Store in Global RAM  DisableCoverage=on  SampleTime=-1
  Difference Inputs1 : Sum  Description=Add in CPU  DisableCoverage=on  Inputs=+-  OutDataTypeStr=Inherit: Inherit via back propagation
  Difference Inputs2 : Sum  Description=Add in CPU  OutDataTypeStr=Inherit: Inherit via back propagation
  FixPt Data Type Duplicate : DataTypeDuplicate  DisableCoverage=on  NumInputPorts=7
  NOT : Logic  Commented=on  Operator=NOT  IconShape=distinctive  AllPortsSameDT=off  OutDataTypeStr=boolean
  NOT1 : Logic  Operator=NOT  IconShape=distinctive  AllPortsSameDT=off  OutDataTypeStr=boolean
  Saturation Dynamic : simulink/Discontinuities/Saturation Dynamic  OutMin=[]  OutMax=[]  OutDataTypeStr=Inherit: Same as second input  OutDataType=fixdt(1, 16)  OutScaling=2^-10  DoSatur=off
  Switch : Switch  Criteria=u2 > Threshold
  Unit Delay : UnitDelay  Commented=on  SampleTime=-1
  delta fall limit : Product  DisableCoverage=on  Inputs=**  OutDataTypeStr=Inherit: Inherit via back propagation  SaturateOnIntegerOverflow=on
  delta rise limit : Product  DisableCoverage=on  Inputs=**  OutDataTypeStr=Inherit: Inherit via back propagation  SaturateOnIntegerOverflow=on
  sample time : SampleTimeMath  DisableCoverage=on  TsampMathOp=Ts Only  weightValue=1
  Y : Outport  InitialOutput=0
  wires:
  up/1 -> delta rise limit/1
  Saturation Dynamic/1 -> FixPt Data Type Duplicate/7, Difference Inputs2/1
  u/1 -> Switch/1, sample time/1, FixPt Data Type Duplicate/5, Difference Inputs1/1
  delta fall limit/1 -> Saturation Dynamic/3, FixPt Data Type Duplicate/3
  delta rise limit/1 -> Saturation Dynamic/1, FixPt Data Type Duplicate/6
  Delay Input2/1 -> FixPt Data Type Duplicate/2, Difference Inputs1/2, Difference Inputs2/2  "Y(k-1)"
  sample time/1 -> delta rise limit/2, delta fall limit/2
  Difference Inputs1/1 -> Saturation Dynamic/2, FixPt Data Type Duplicate/4  "( U(k) - Y(k-1) )"
  Difference Inputs2/1 -> Switch/3, FixPt Data Type Duplicate/1, Y/1
  lo/1 -> delta fall limit/1
  Switch/1 -> Delay Input2/1
  NOT1/1 -> Switch/2
  ? -> Unit Delay/1, AND/1
  Unit Delay/1 -> NOT/1
  NOT/1 -> AND/2
  Enable/1 -> NOT1/1

== system Lib_Piccolo/Throttle Control (Alt Mode)/Speed Flags/CAS2TAS ==
  Feedback Bus : Inport
  CAS : Inport  Port=2
  Bus Selector2 : BusSelector  OutputSignals=airDensity_kgm
  Constant : Constant  Value=1.225
  Divide : Product  Inputs=*/
  Multiply : Product
  Sqrt : Sqrt  SaturateOnIntegerOverflow=on
  TAS : Outport
  wires:
  CAS/1 -> Multiply/1
  Multiply/1 -> TAS/1
  Divide/1 -> Sqrt/1
  Sqrt/1 -> Multiply/2
  Constant/1 -> Divide/1
  Feedback Bus/1 -> Bus Selector2/1
  Bus Selector2/1 -> Divide/2  "<airDensity_kgm>"

== system Lib_Piccolo/Throttle Control (Alt Mode)/Speed Flags/CAS2TAS1 ==
  Feedback Bus : Inport
  CAS : Inport  Port=2
  Bus Selector2 : BusSelector  OutputSignals=airDensity_kgm
  Constant : Constant  Value=1.225
  Divide : Product  Inputs=*/
  Multiply : Product
  Sqrt : Sqrt  SaturateOnIntegerOverflow=on
  TAS : Outport
  wires:
  CAS/1 -> Multiply/1
  Multiply/1 -> TAS/1
  Divide/1 -> Sqrt/1
  Sqrt/1 -> Multiply/2
  Constant/1 -> Divide/1
  Feedback Bus/1 -> Bus Selector2/1
  Bus Selector2/1 -> Divide/2  "<airDensity_kgm>"

== system Lib_Piccolo/WOW Archive Container/Load Cell WoW Model 10/Subsystem ==
  note: Ground Detection Logic
  Sim.WOW_NG_N : Inport
  Sim.WOW_L_N : Inport  Port=2
  RESET : Inport  Port=3
  Sim.WOW_R_N : Inport  Port=4
  PICCOLO_AP_MODE : Inport  Port=5
  Bus Creator1 : BusCreator  Inputs=6
  Compare To Constant1 : simulink/Logic and Bit Operations/Compare To Constant  relop===  const=0  OutDataTypeStr=uint8
  Compare To Constant6 : simulink/Logic and Bit Operations/Compare To Constant  relop=>=  const=4  OutDataTypeStr=uint8
  LPF L : Subsystem  mask{Cutoff=SensorModel.WOW.Cell.fc, Init=0}
      mask prompts: Cutoff "Cutoff Frequency [Hz]"; Init "Initial Condition"
  LPF N : Subsystem  mask{Cutoff=SensorModel.WOW.Cell.fc, Init=0}
      mask prompts: Cutoff "Cutoff Frequency [Hz]"; Init "Initial Condition"
  LPF R : Subsystem  mask{Cutoff=SensorModel.WOW.Cell.fc, Init=0}
      mask prompts: Cutoff "Cutoff Frequency [Hz]"; Init "Initial Condition"
  Landing Configuration : Subsystem
  OR : Logic  Operator=OR  IconShape=distinctive  AllPortsSameDT=off  OutDataTypeStr=boolean
  Saturation : Saturate  UpperLimit=SensorModel.WOW.Cell.SaturationUpper  LowerLimit=SensorModel.WOW.Cell.SaturationLower
  Saturation1 : Saturate  UpperLimit=SensorModel.WOW.Cell.SaturationUpper  LowerLimit=SensorModel.WOW.Cell.SaturationLower
  Saturation2 : Saturate  UpperLimit=SensorModel.WOW.Cell.SaturationUpper  LowerLimit=SensorModel.WOW.Cell.SaturationLower
  Switch : Switch  Criteria=u2 > Threshold
  T/O Configuration : Subsystem
  Sim.WOW_Filt_NG : Outport
  Sim.WOW_Filt_L : Outport  Port=2
  Contact : Outport  Port=3
  Sim.WOW_Filt_R : Outport  Port=4
  wires:
  Saturation2/1 -> LPF R/1(Input)
  Saturation1/1 -> LPF L/1(Input)
  Saturation/1 -> LPF N/1(Input)
  Sim.WOW_R_N/1 -> Bus Creator1/6, Saturation2/1
  Switch/1 -> Contact/1
  OR/1 -> Switch/2
  T/O Configuration/1(ContactBool) -> Switch/3
  Compare To Constant1/1 -> OR/2
  LPF N/1(Output) -> Bus Creator1/1, Sim.WOW_Filt_NG/1  "Sim.WOW_Filt_NG"
  Landing Configuration/1(ContactBool) -> Switch/1
  Sim.WOW_NG_N/1 -> Bus Creator1/4, Saturation/1
  RESET/1 -> LPF R/2(Reset), LPF L/2(Reset), LPF N/2(Reset)
  Sim.WOW_L_N/1 -> Bus Creator1/5, Saturation1/1
  LPF L/1(Output) -> Bus Creator1/2, Sim.WOW_Filt_L/1  "Sim.WOW_Filt_L"
  Bus Creator1/1 -> Landing Configuration/1(Sim.WOW_Filt), T/O Configuration/1(Sim.WOW_Filt)
  Compare To Constant6/1 -> OR/1
  PICCOLO_AP_MODE/1 -> Compare To Constant6/1, Compare To Constant1/1
  LPF R/1(Output) -> Bus Creator1/3, Sim.WOW_Filt_R/1  "Sim.WOW_Filt_R"

== system Lib_Piccolo/WOW Archive Container/Load Cell WoW Model 10_OLD/Subsystem ==
  note: Ground Detection Logic
  Sim.WOW_NG_N : Inport
  Sim.WOW_L_N : Inport  Port=2
  RESET : Inport  Port=3
  Sim.WOW_R_N : Inport  Port=4
  PICCOLO_AP_MODE : Inport  Port=5
  Bus Creator1 : BusCreator  Inputs=3
  Bus Creator2 : BusCreator  Inputs=3
  Compare To Constant1 : simulink/Logic and Bit Operations/Compare To Constant  relop===  const=0  OutDataTypeStr=uint8
  Compare To Constant6 : simulink/Logic and Bit Operations/Compare To Constant  relop=>=  const=4  OutDataTypeStr=uint8
  LPF L : Subsystem  mask{Cutoff=SensorModel.WOW.Cell.fc, Init=0}
      mask prompts: Cutoff "Cutoff Frequency [Hz]"; Init "Initial Condition"
  LPF N : Subsystem  mask{Cutoff=SensorModel.WOW.Cell.fc, Init=0}
      mask prompts: Cutoff "Cutoff Frequency [Hz]"; Init "Initial Condition"
  LPF R : Subsystem  mask{Cutoff=SensorModel.WOW.Cell.fc, Init=0}
      mask prompts: Cutoff "Cutoff Frequency [Hz]"; Init "Initial Condition"
  Landing Configuration : Subsystem
  OR : Logic  Operator=OR  IconShape=distinctive  AllPortsSameDT=off  OutDataTypeStr=boolean
  Switch : Switch  Criteria=u2 > Threshold
  T/O Configuration : Subsystem
  Sim.WOW_Filt_NG : Outport
  Sim.WOW_Filt_L : Outport  Port=2
  Contact : Outport  Port=3
  Sim.WOW_Filt_R : Outport  Port=4
  wires:
  LPF R/1(Output) -> Sim.WOW_Filt_R/1, Bus Creator1/3  "Sim.WOW_Filt_R"
  PICCOLO_AP_MODE/1 -> Compare To Constant1/1, Compare To Constant6/1
  Compare To Constant6/1 -> OR/1
  Bus Creator1/1 -> T/O Configuration/1(Sim.WOW_Filt), Landing Configuration/1(Sim.WOW_Filt)
  LPF L/1(Output) -> Sim.WOW_Filt_L/1, Bus Creator1/2  "Sim.WOW_Filt_L"
  Sim.WOW_L_N/1 -> Bus Creator2/2, LPF L/1(Input)  "WOW_L"
  RESET/1 -> LPF N/2(Reset), LPF L/2(Reset), LPF R/2(Reset)
  Sim.WOW_NG_N/1 -> Bus Creator2/1, LPF N/1(Input)  "WOW_NG"
  Landing Configuration/1(ContactBool) -> Switch/1
  LPF N/1(Output) -> Sim.WOW_Filt_NG/1, Bus Creator1/1  "Sim.WOW_Filt_NG"
  Compare To Constant1/1 -> OR/2
  T/O Configuration/1(ContactBool) -> Switch/3
  OR/1 -> Switch/2
  Switch/1 -> Contact/1
  Sim.WOW_R_N/1 -> Bus Creator2/3, LPF R/1(Input)  "WOW_R"
  Bus Creator2/1 -> Landing Configuration/2(Sim.WOW)

== system Lib_Piccolo/WOW Archive Container/Load Cell WoW Model 11/Subsystem ==
  note: Ground Detection Logic
  Sim.WOW_NG_N : Inport
  Sim.WOW_L_N : Inport  Port=2
  RESET : Inport  Port=3
  Sim.WOW_R_N : Inport  Port=4
  PICCOLO_AP_MODE : Inport  Port=5
  Bus Creator1 : BusCreator  Inputs=6
  Compare To Constant1 : simulink/Logic and Bit Operations/Compare To Constant  relop===  const=0  OutDataTypeStr=uint8
  Compare To Constant6 : simulink/Logic and Bit Operations/Compare To Constant  relop=>=  const=4  OutDataTypeStr=uint8
  LPF L : Subsystem  mask{Cutoff=SensorModel.WOW.Cell.fc, Init=0}
      mask prompts: Cutoff "Cutoff Frequency [Hz]"; Init "Initial Condition"
  LPF N : Subsystem  mask{Cutoff=SensorModel.WOW.Cell.fc, Init=0}
      mask prompts: Cutoff "Cutoff Frequency [Hz]"; Init "Initial Condition"
  LPF R : Subsystem  mask{Cutoff=SensorModel.WOW.Cell.fc, Init=0}
      mask prompts: Cutoff "Cutoff Frequency [Hz]"; Init "Initial Condition"
  Landing Configuration : Subsystem
  OR : Logic  Operator=OR  IconShape=distinctive  AllPortsSameDT=off  OutDataTypeStr=boolean
  Saturation : Saturate  UpperLimit=SensorModel.WOW.Cell.SaturationUpper  LowerLimit=SensorModel.WOW.Cell.SaturationLower
  Saturation1 : Saturate  UpperLimit=SensorModel.WOW.Cell.SaturationUpper  LowerLimit=SensorModel.WOW.Cell.SaturationLower
  Saturation2 : Saturate  UpperLimit=SensorModel.WOW.Cell.SaturationUpper  LowerLimit=SensorModel.WOW.Cell.SaturationLower
  Switch : Switch  Criteria=u2 > Threshold
  T/O Configuration : Subsystem
  Sim.WOW_Filt_NG : Outport
  Sim.WOW_Filt_L : Outport  Port=2
  Contact : Outport  Port=3
  Sim.WOW_Filt_R : Outport  Port=4
  wires:
  LPF R/1(Output) -> Sim.WOW_Filt_R/1, Bus Creator1/3  "Sim.WOW_Filt_R"
  PICCOLO_AP_MODE/1 -> Compare To Constant1/1, Compare To Constant6/1
  Compare To Constant6/1 -> OR/1
  Bus Creator1/1 -> T/O Configuration/1(Sim.WOW_Filt), Landing Configuration/1(Sim.WOW_Filt)
  LPF L/1(Output) -> Sim.WOW_Filt_L/1, Bus Creator1/2  "Sim.WOW_Filt_L"
  Sim.WOW_L_N/1 -> Saturation1/1, Bus Creator1/5
  RESET/1 -> LPF N/2(Reset), LPF L/2(Reset), LPF R/2(Reset)
  Sim.WOW_NG_N/1 -> Saturation/1, Bus Creator1/4
  Landing Configuration/1(ContactBool) -> Switch/1
  LPF N/1(Output) -> Sim.WOW_Filt_NG/1, Bus Creator1/1  "Sim.WOW_Filt_NG"
  Compare To Constant1/1 -> OR/2
  T/O Configuration/1(ContactBool) -> Switch/3
  OR/1 -> Switch/2
  Switch/1 -> Contact/1
  Sim.WOW_R_N/1 -> Saturation2/1, Bus Creator1/6
  Saturation/1 -> LPF N/1(Input)
  Saturation1/1 -> LPF L/1(Input)
  Saturation2/1 -> LPF R/1(Input)
